simulink model "rlWalkingBipedRobot"  (R2024a)
settings: Solver=ode23t  StartTime=0.0  StopTime=Tf  RelTol=1e-2  EnableMultiTasking=on
values from neighbouring files (symbols this model uses):
  height_plane = 0.025    [robotParametersRL.m]
  init_angs_L = zeros(1,2)    [robotParametersRL.m]    (also in walkerResetFcn.m)
  init_angs_R = zeros(1,2)    [robotParametersRL.m]    (also in walkerResetFcn.m)
  init_height = foot_z + h +                torso_z/2 + torso_offset_z + height_plane/2    (= 21.0125)    [robotParametersRL.m]
  joint_stiffness = 0    [robotParametersRL.m]
  lower_leg_length = 10    [robotParametersRL.m]
  max_torque = 3    [robotParametersRL.m]
  plane_x = 25    [robotParametersRL.m]
  plane_y = 10    [robotParametersRL.m]
  s = load(files(i).name,'trainingStats')    [comparePerformance.m]
  Tf = 10    [robotParametersRL.m]
  torso_offset_x = -1    [robotParametersRL.m]
  torso_offset_z = -2    [robotParametersRL.m]
  torso_x = 5    [robotParametersRL.m]
  torso_y = 8    [robotParametersRL.m]
  torso_z = 8    [robotParametersRL.m]
  Ts = 0.025    [robotParametersRL.m]
  upper_leg_length = 10    [robotParametersRL.m]
  wx0 = 0    [robotParametersRL.m]
  wy0 = 0    [robotParametersRL.m]
undefined symbols (not defined in the file or in its folder): X, Y, Z
libraries: sm_lib x27, nesl_utility x14, walkingRobotUtils x10, simulink x5, rllib x1
settings Model: Creator=The MathWorks, Inc.  LastModifiedBy=Administrator
settings SolverCC: ZeroCrossAlgorithm=Adaptive  AlgebraicLoopSolver=TrustRegion
settings DataIOCC: SaveOutput=off  SignalLogging=off  DSMLogging=off  SaveTime=off  ReturnWorkspaceOutputs=off  OutputTimes=0:0.01:10
settings OptimizationCC: LifeSpan=inf
settings DebuggingCC: MaxConsecutiveZCsMsg=warning  IgnoredZcDiagnostic=none  UnconnectedInputMsg=warning  UnconnectedOutputMsg=warning  UnconnectedLineMsg=warning  AllowSymbolicDim=off  SFUnexpectedBacktrackingDiag=warning  SFNoUnconditionalDefaultTransitionDiag=warning  SFExecutionAtInitializationDiag=none  UnitsInconsistencyMsg=none  ArithmeticOperatorsInVariantConditions=warning
settings ModelReferenceCC: EnableRefExpFcnMdlSchedulingChecks=on
settings SFSimCC: SimUseLocalCustomCode=off  CustomCodeUndefinedFunction=UseInterfaceOnly
settings RTWCC: RTWUseLocalCustomCode=off  GPUComputeCapability=3.5
settings CodeAppCC: StateflowObjectComments=on
settings GRTTargetCC: TargetLangStandard=C89/C90 (ANSI)
settings ConfigComp: CovMetricSettings=dw  CovSaveCumulativeToWorkspaceVar=on  CovSaveSingleToWorkspaceVar=on  CovExternalEMLEnable=off  CovSFcnEnable=off
settings SimscapeCC: SimscapeNormalizeSystem=off  SimscapeLogOpenViewer=on  SimscapeLogLimitData=off  SimscapeLogDataHistory=10000
settings ConfigurationSet: Description=SimMechanics 2G
settings DiagnosticsConfigSet: SimMechanicsRigidlyBoundBlock=none
settings ExplorerConfigSet: InternalSimMechanicsExplorerSettings="<ExplorerConfiguration><canonicalview>default</canonicalview><AnimationSetting><BasePlaybackSpeed>1.0</BasePlaybackSpeed><PlaybackSpeedFactor>1.0</PlaybackSpeedFactor></AnimationSetting><TilePanel><TileInfo><Tiles Columns=\"1\" Count=\"1\" Rows=\"1\"><Column Weight=\"1\"/><Row Weight=\"1\"/><Tile Height=\"1\" Width=\"1\" X=\"0\" Y=\"0\"/></Tiles></TileInfo><SceneInfo><SceneViewer><BGColor><R>0.60000002384185791</R><G>0.60000002384185791</G><B>0.60000002384185791</B></BGColor><Camera><DoPerspective>off</DoPerspective><Position><X>7.18002534815406079</X><Y>-8.21011991112170847</Y><Z>8.33180938462712462</Z></Position><Center><X>1.10741005252516134</X><Y>-0.176829942633513204</Y><Z>0.646464709811595872</Z></Center><Up><X>-0.335329266167064488</X><Y>0.506481739462631531</Y><Z>0.79437430147428989</Z></Up><ViewLimDist>1</ViewLimDist><YLim>0.739205014828661411</YLim><XLim>1.12849377732657596</XLim></Camera></SceneViewer></SceneInfo></TilePanel><MechEditorPanel><Cameras/><GfxPanelCameraMap/><VideoCreator><PlaybackSpeedRatio>1.0</PlaybackSpeedRatio><FrameRate>30</FrameRate><VideoFormat>Motion JPEG AVI</VideoFormat><FrameSize>auto</FrameSize></VideoCreator></MechEditorPanel></ExplorerConfiguration>"

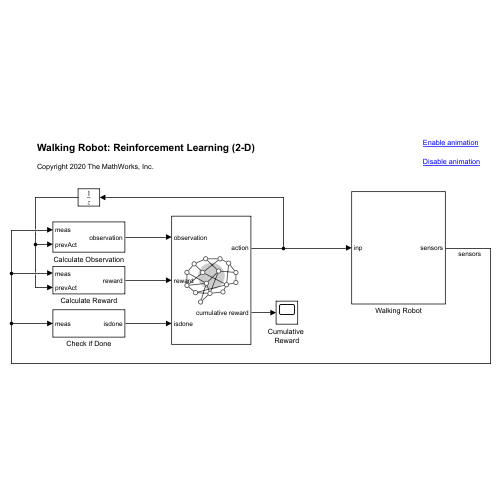
[thumbnail: Simulink's stored preview of the top-level diagram]
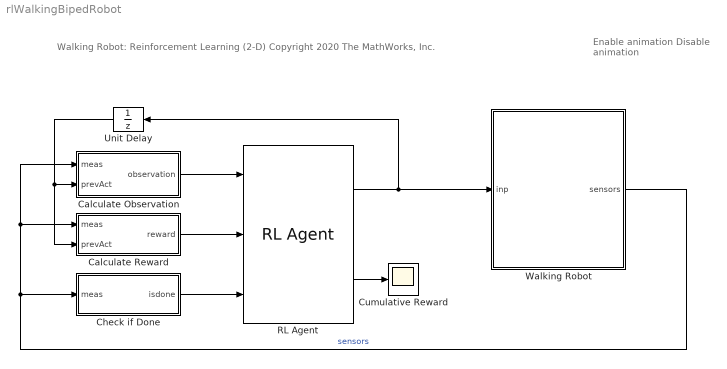
== system rlWalkingBipedRobot ==
  note: Enable animation
      |
      | Disable animation
  note: Walking Robot: Reinforcement Learning (2-D)
      |
      | Copyright 2020 The MathWorks, Inc.
  Calculate Observation : Subsystem
  Calculate Reward : Subsystem
  Check if Done : Subsystem
  Cumulative Reward : Scope
  RL Agent : rllib/RL Agent  Agent=agent  ExternalActionAsInput=off  ProvideLastAction=off  ProvideCumRwd=on  TreatAsDirectFeedthrough=on  UseStrictObservationDataTypes=off
  Unit Delay : UnitDelay  SampleTime=-1  HasFrameUpgradeWarning=on
  Walking Robot : Subsystem
  wires:
  Walking Robot/1(sensors) -> Calculate Reward/1(meas), Calculate Observation/1(meas), Check if Done/1(meas)  "sensors"
  Calculate Reward/1(reward) -> RL Agent/2
  Calculate Observation/1(observation) -> RL Agent/1
  Check if Done/1(isdone) -> RL Agent/3
  RL Agent/2 -> Cumulative Reward/1
  Unit Delay/1 -> Calculate Reward/2(prevAct), Calculate Observation/2(prevAct)
  RL Agent/1 -> Walking Robot/1(inp), Unit Delay/1

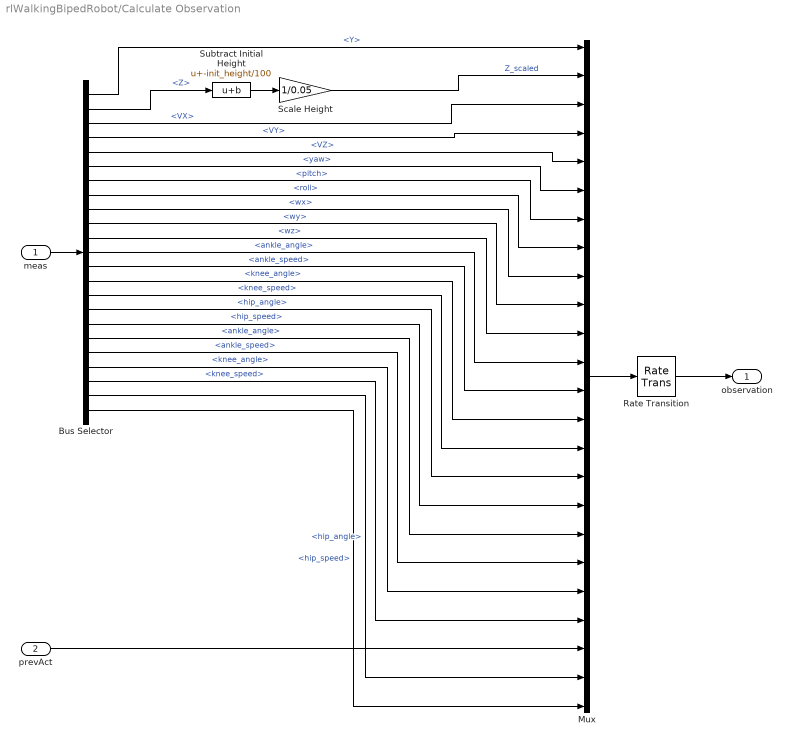
== system rlWalkingBipedRobot/Calculate Observation ==
  meas : Inport
  prevAct : Inport  Port=2
  Bus Selector : BusSelector  OutputSignals=Y,Z,VX,VY,VZ,yaw,pitch,roll,wx,wy,wz,measR.ankle_angle,measR.ankle_speed,measR.knee_angle,measR.knee_speed,measR.hip_angle,measR.hip_speed,measL.ankle_angle,measL.ankle_speed,measL.knee_angle,measL.knee_speed,measL.hip_angle,measL.hip_speed
  Mux : Mux  Inputs=24
  Rate Transition : RateTransition
  Scale Height : Gain  Gain=1/0.05
  Subtract Initial Height : Bias  Bias=-init_height/100  SaturateOnIntegerOverflow=off
  observation : Outport  VectorParamsAs1DForOutWhenUnconnected=off
  wires:
  meas/1 -> Bus Selector/1
  Mux/1 -> Rate Transition/1
  Rate Transition/1 -> observation/1
  prevAct/1 -> Mux/22
  Bus Selector/2 -> Subtract Initial Height/1  "<Z>"
  Subtract Initial Height/1 -> Scale Height/1
  Scale Height/1 -> Mux/2  "Z_scaled"
  Bus Selector/1 -> Mux/1  "<Y>"
  Bus Selector/4 -> Mux/4  "<VY>"
  Bus Selector/5 -> Mux/5  "<VZ>"
  Bus Selector/3 -> Mux/3  "<VX>"
  Bus Selector/6 -> Mux/6  "<yaw>"
  Bus Selector/7 -> Mux/7  "<pitch>"
  Bus Selector/8 -> Mux/8  "<roll>"
  Bus Selector/9 -> Mux/9  "<wx>"
  Bus Selector/10 -> Mux/10  "<wy>"
  Bus Selector/11 -> Mux/11  "<wz>"
  Bus Selector/12 -> Mux/12  "<ankle_angle>"
  Bus Selector/13 -> Mux/13  "<ankle_speed>"
  Bus Selector/14 -> Mux/14  "<knee_angle>"
  Bus Selector/15 -> Mux/15  "<knee_speed>"
  Bus Selector/16 -> Mux/16  "<hip_angle>"
  Bus Selector/17 -> Mux/17  "<hip_speed>"
  Bus Selector/18 -> Mux/18  "<ankle_angle>"
  Bus Selector/19 -> Mux/19  "<ankle_speed>"
  Bus Selector/20 -> Mux/20  "<knee_angle>"
  Bus Selector/21 -> Mux/21  "<knee_speed>"
  Bus Selector/22 -> Mux/23  "<hip_angle>"
  Bus Selector/23 -> Mux/24  "<hip_speed>"

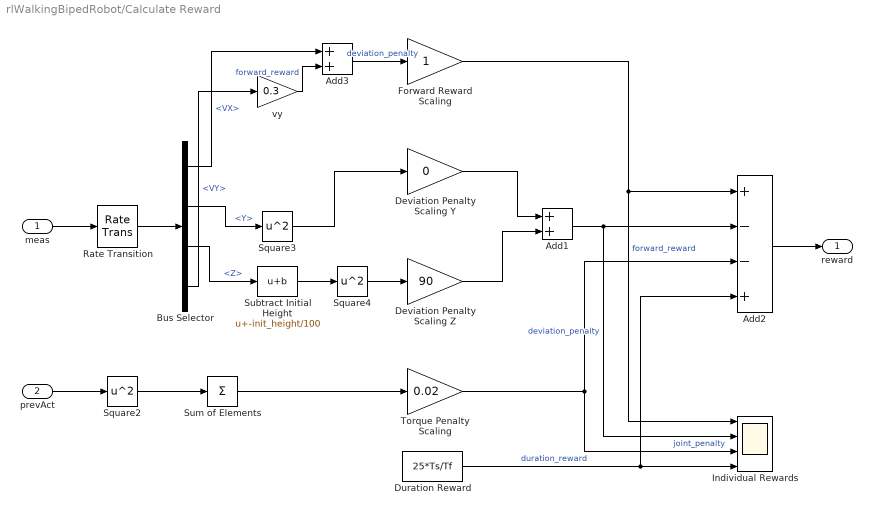
== system rlWalkingBipedRobot/Calculate Reward ==
  meas : Inport
  prevAct : Inport  Port=2
  Add1 : Sum
  Add2 : Sum  Inputs=+--+
  Add3 : Sum
  Bus Selector : BusSelector  OutputSignals=VX,Y,Z,VY
  Deviation Penalty Scaling Y : Gain  Gain=0
  Deviation Penalty Scaling Z : Gain  Gain=90
  Duration Reward : Constant  Value=25*Ts/Tf
  Forward Reward Scaling : Gain
  Individual Rewards : Scope  NumInputPorts=4
  Rate Transition : RateTransition  OutPortSampleTime=Ts
  Square2 : Math  Operator=square  SignedPower=on
  Square3 : Math  Operator=square  SignedPower=on
  Square4 : Math  Operator=square  SignedPower=on
  Subtract Initial Height : Bias  Bias=-init_height/100  SaturateOnIntegerOverflow=off
  Sum of Elements : Sum  Inputs=+
  Torque Penalty Scaling : Gain  Gain=0.02
  vy : Gain  Gain=0.3
  reward : Outport  VectorParamsAs1DForOutWhenUnconnected=off
  wires:
  meas/1 -> Rate Transition/1
  Rate Transition/1 -> Bus Selector/1
  Add2/1 -> reward/1
  Add1/1 -> Add2/2, Individual Rewards/2  "deviation_penalty"
  Forward Reward Scaling/1 -> Add2/1, Individual Rewards/1  "forward_reward"
  Sum of Elements/1 -> Torque Penalty Scaling/1
  Bus Selector/1 -> Add3/1  "<VX>"
  Bus Selector/2 -> Square3/1  "<Y>"
  Square3/1 -> Deviation Penalty Scaling Y/1
  Duration Reward/1 -> Individual Rewards/4, Add2/4  "duration_reward"
  prevAct/1 -> Square2/1
  Square2/1 -> Sum of Elements/1
  Torque Penalty Scaling/1 -> Add2/3, Individual Rewards/3  "joint_penalty"
  Square4/1 -> Deviation Penalty Scaling Z/1
  Bus Selector/3 -> Subtract Initial Height/1  "<Z>"
  Subtract Initial Height/1 -> Square4/1
  Deviation Penalty Scaling Z/1 -> Add1/2
  Deviation Penalty Scaling Y/1 -> Add1/1
  Add3/1 -> Forward Reward Scaling/1  "deviation_penalty"
  vy/1 -> Add3/2  "forward_reward"
  Bus Selector/4 -> vy/1  "<VY>"

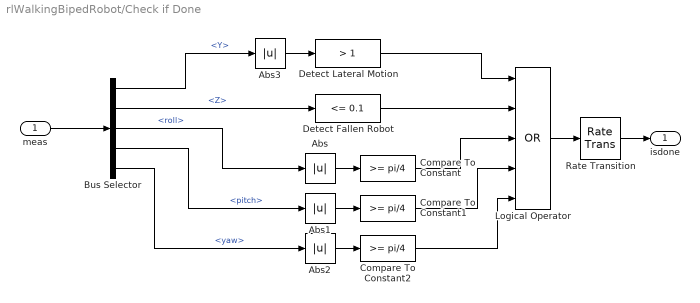
== system rlWalkingBipedRobot/Check if Done ==
  meas : Inport
  Abs{,1..3} (4 alike) : Abs  SaturateOnIntegerOverflow=off
  Bus Selector : BusSelector  OutputSignals=Y,Z,roll,pitch,yaw
  Compare To Constant : simulink/Logic and Bit Operations/Compare To Constant  relop=>=  const=pi/4  OutDataTypeStr=boolean
  Compare To Constant1 : simulink/Logic and Bit Operations/Compare To Constant  relop=>=  const=pi/4  OutDataTypeStr=boolean
  Compare To Constant2 : simulink/Logic and Bit Operations/Compare To Constant  relop=>=  const=pi/4  OutDataTypeStr=boolean
  Detect Fallen Robot : simulink/Logic and Bit Operations/Compare To Constant  relop=<=  const=0.1  OutDataTypeStr=boolean
  Detect Lateral Motion : simulink/Logic and Bit Operations/Compare To Constant  relop=>  const=1  OutDataTypeStr=boolean
  Logical Operator : Logic  Operator=OR  Inputs=5  AllPortsSameDT=off  OutDataTypeStr=boolean
  Rate Transition : RateTransition
  isdone : Outport  VectorParamsAs1DForOutWhenUnconnected=off
  wires:
  Logical Operator/1 -> Rate Transition/1
  Bus Selector/2 -> Detect Fallen Robot/1  "<Z>"
  meas/1 -> Bus Selector/1
  Detect Fallen Robot/1 -> Logical Operator/2
  Bus Selector/3 -> Abs/1  "<roll>"
  Bus Selector/4 -> Abs1/1  "<pitch>"
  Compare To Constant/1 -> Logical Operator/3
  Abs/1 -> Compare To Constant/1
  Abs1/1 -> Compare To Constant1/1
  Compare To Constant1/1 -> Logical Operator/4
  Rate Transition/1 -> isdone/1
  Abs2/1 -> Compare To Constant2/1
  Bus Selector/5 -> Abs2/1  "<yaw>"
  Compare To Constant2/1 -> Logical Operator/5
  Abs3/1 -> Detect Lateral Motion/1
  Bus Selector/1 -> Abs3/1  "<Y>"
  Detect Lateral Motion/1 -> Logical Operator/1

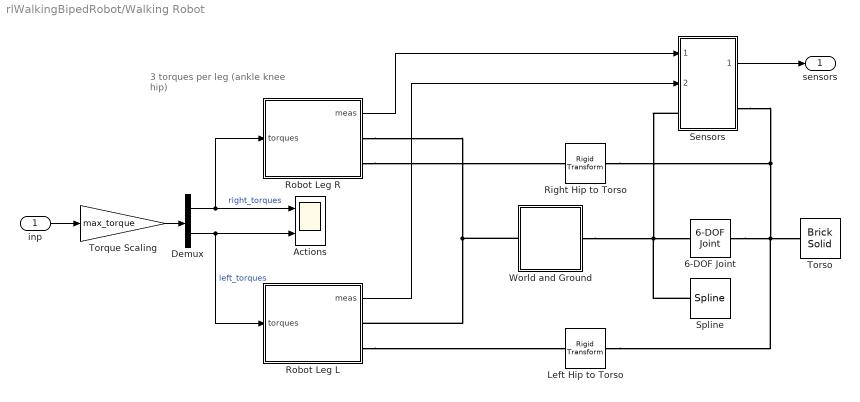
== system rlWalkingBipedRobot/Walking Robot ==
  note: 3 torques per leg
      | (ankle knee hip)
  inp : Inport
  6-DOF Joint : sm_lib/Joints/6-DOF Joint  JointMode=Normal  CompositeWrenchDir=FollowerOnBase  CompositeWrenchFrame=BaseFrame  SenseConstraintForce=off  SenseConstraintTorque=off  SenseTotalForce=off  SenseTotalTorque=off  PxPositionTargetSpecify=on  PxPositionTargetPriority=High  PxPositionTargetValue=0  PxPositionTargetValueUnits=m  PxVelocityTargetSpecify=on  PxVelocityTargetPriority=High  PxVelocityTargetValue=vx0  PxVelocityTargetValueUnits=m/s  PxEquilibriumPosition=0  PxEquilibriumPositionUnits=m  PxSpringStiffness=0  PxSpringStiffnessUnits=N/m  PxDampingCoefficient=world_damping  PxDampingCoefficientUnits=N/(m/s)  PxLowerLimitSpecify=off  PxLowerLimitBound=-1  PxLowerLimitBoundUnits=m  PxLowerLimitStiffness=1e6  PxLowerLimitStiffnessUnits=N/m  PxLowerLimitDamping=1e3  PxLowerLimitDampingUnits=N/(m/s)  PxLowerLimitTransitionRegionWidth=1e-4  PxLowerLimitTransitionRegionWidthUnits=m  PxUpperLimitSpecify=off  PxUpperLimitBound=1  PxUpperLimitBoundUnits=m  PxUpperLimitStiffness=1e6  PxUpperLimitStiffnessUnits=N/m  PxUpperLimitDamping=1e3  PxUpperLimitDampingUnits=N/(m/s)  PxUpperLimitTransitionRegionWidth=1e-4  PxUpperLimitTransitionRegionWidthUnits=m  PxTorqueActuationMode=NoTorque  PxMotionActuationMode=ComputedMotion  PxSensePosition=off  PxSenseVelocity=off  PxSenseAcceleration=off  PxSenseTorqueForce=off  PxSenseLowerLimitTorqueForce=off  PxSenseUpperLimitTorqueForce=off  PyPositionTargetSpecify=on  PyPositionTargetPriority=High  PyPositionTargetValue=0  PyPositionTargetValueUnits=m  PyVelocityTargetSpecify=on  PyVelocityTargetPriority=High  PyVelocityTargetValue=0  PyVelocityTargetValueUnits=m/s  PyEquilibriumPosition=0  PyEquilibriumPositionUnits=m  PySpringStiffness=0  PySpringStiffnessUnits=N/m  PyDampingCoefficient=world_damping  PyDampingCoefficientUnits=N/(m/s)  PyLowerLimitSpecify=off  PyLowerLimitBound=-1  PyLowerLimitBoundUnits=m  PyLowerLimitStiffness=1e6  PyLowerLimitStiffnessUnits=N/m  PyLowerLimitDamping=1e3  PyLowerLimitDampingUnits=N/(m/s)  PyLowerLimitTransitionRegionWidth=1e-4  PyLowerLimitTransitionRegionWidthUnits=m  PyUpperLimitSpecify=off  PyUpperLimitBound=1  PyUpperLimitBoundUnits=m  PyUpperLimitStiffness=1e6  PyUpperLimitStiffnessUnits=N/m  PyUpperLimitDamping=1e3  PyUpperLimitDampingUnits=N/(m/s)  PyUpperLimitTransitionRegionWidth=1e-4  PyUpperLimitTransitionRegionWidthUnits=m  PyTorqueActuationMode=NoTorque  PyMotionActuationMode=ComputedMotion  PySensePosition=off  PySenseVelocity=off  PySenseAcceleration=off  PySenseTorqueForce=off  PySenseLowerLimitTorqueForce=off  PySenseUpperLimitTorqueForce=off  PzPositionTargetSpecify=on  PzPositionTargetPriority=High  PzPositionTargetValue=init_height  PzPositionTargetValueUnits=cm  PzVelocityTargetSpecify=off  PzVelocityTargetPriority=High  PzVelocityTargetValue=0  PzVelocityTargetValueUnits=m/s  PzEquilibriumPosition=0  PzEquilibriumPositionUnits=m  PzSpringStiffness=0  PzSpringStiffnessUnits=N/m  PzDampingCoefficient=world_damping  PzDampingCoefficientUnits=N/(m/s)  PzLowerLimitSpecify=off  PzLowerLimitBound=-1  PzLowerLimitBoundUnits=m  PzLowerLimitStiffness=1e6  PzLowerLimitStiffnessUnits=N/m  PzLowerLimitDamping=1e3  PzLowerLimitDampingUnits=N/(m/s)  PzLowerLimitTransitionRegionWidth=1e-4  PzLowerLimitTransitionRegionWidthUnits=m  PzUpperLimitSpecify=off  PzUpperLimitBound=1  PzUpperLimitBoundUnits=m  PzUpperLimitStiffness=1e6  PzUpperLimitStiffnessUnits=N/m  PzUpperLimitDamping=1e3  PzUpperLimitDampingUnits=N/(m/s)  PzUpperLimitTransitionRegionWidth=1e-4  PzUpperLimitTransitionRegionWidthUnits=m  PzTorqueActuationMode=NoTorque  PzMotionActuationMode=ComputedMotion  PzSensePosition=off  PzSenseVelocity=off  PzSenseAcceleration=off  PzSenseTorqueForce=off  PzSenseLowerLimitTorqueForce=off  PzSenseUpperLimitTorqueForce=off  SphPositionTargetSpecify=on  SphPositionTargetPriority=High  SphPositionTargetRotationMethod=RotationSequence  SphPositionTargetFollAlignAxisA=+X  SphPositionTargetBaseAlignAxisA=+Y  SphPositionTargetFollAlignAxisB=+Y  SphPositionTargetBaseAlignAxisB=+Z  SphPositionTargetRotationStandardAxis=+Z  SphPositionTargetRotationAngle=0.0  SphPositionTargetRotationAngleUnits=deg  SphPositionTargetRotationArbitraryAxis=[0 0 1]  SphPositionTargetRotationSequenceAxes=FollowerAxes  SphPositionTargetRotationSequence=XYX  SphPositionTargetRotationSequenceAngles=[wx0 wy0 0]  SphPositionTargetRotationSequenceAnglesUnits=rad  SphPositionTargetRotationMatrix=eye(3)  SphPositionTargetQuaternion=[1 0 0 0]  SphVelocityTargetSpecify=off  SphVelocityTargetPriority=High  SphVelocityTargetValue=[0 0 0]  SphVelocityTargetValueUnits=deg/s  SphVelocityTargetInFollowerFrame=on  SphEqPosRotationMethod=None  SphEqPosFollAlignAxisA=+X  SphEqPosBaseAlignAxisA=+Y  SphEqPosFollAlignAxisB=+Y  SphEqPosBaseAlignAxisB=+Z  SphEqPosRotationStandardAxis=+Z  SphEqPosRotationAngle=0.0  SphEqPosRotationAngleUnits=deg  SphEqPosRotationArbitraryAxis=[0 0 1]  SphEqPosRotationSequenceAxes=FollowerAxes  SphEqPosRotationSequence=XYX  SphEqPosRotationSequenceAngles=[0 0 0]  SphEqPosRotationSequenceAnglesUnits=deg  SphEqPosRotationMatrix=[1 0 0; 0 1 0; 0 0 1]  SphEqPosQuaternion=[1 0 0 0]  SphSpringStiffness=0  SphSpringStiffnessUnits=N*m/deg  SphDampingCoefficient=world_rot_damping  SphDampingCoefficientUnits=N*m/(rad/s)  SphLowerLimitSpecify=off  SphLowerLimitBound=15  SphLowerLimitBoundUnits=deg  SphLowerLimitStiffness=1e4  SphLowerLimitStiffnessUnits=N*m/deg  SphLowerLimitDamping=10  SphLowerLimitDampingUnits=N*m/(deg/s)  SphLowerLimitTransitionRegionWidth=0.1  SphLowerLimitTransitionRegionWidthUnits=deg  SphUpperLimitSpecify=off  SphUpperLimitBound=45  SphUpperLimitBoundUnits=deg  SphUpperLimitStiffness=1e4  SphUpperLimitStiffnessUnits=N*m/deg  SphUpperLimitDamping=10  SphUpperLimitDampingUnits=N*m/(deg/s)  SphUpperLimitTransitionRegionWidth=0.1  SphUpperLimitTransitionRegionWidthUnits=deg  SphTorqueActuationMode=NoTorque  SphActuateTorqueX=off  SphActuateTorqueY=off  SphActuateTorqueZ=off  SphActuateTorque=off  SphActuationFrame=BaseFrame  SphSensePosition=off  SphSenseVelocityX=off  SphSenseVelocityY=off  SphSenseVelocityZ=off  SphSenseVelocity=off  SphSenseAccelerationX=off  SphSenseAccelerationY=off  SphSenseAccelerationZ=off  SphSenseAcceleration=off  SphSenseLowerLimitTorqueMag=off  SphSenseUpperLimitTorqueMag=off  SphSensingFrame=BaseFrame
  Actions : Scope  NumInputPorts=2
  Demux : Demux  Outputs=2
  Left Hip to Torso : sm_lib/Frames and Transforms/Rigid Transform  RotationMethod=None  FollAlignAxisA=+X  BaseAlignAxisA=+Y  FollAlignAxisB=+Y  BaseAlignAxisB=+Z  RotationStandardAxis=+Z  RotationAngle=0.0  RotationAngleUnits=deg  RotationArbitraryAxis=[0 0 1]  RotationSequenceAxes=FollowerAxes  RotationSequence=XYX  RotationSequenceAngles=[0 0 0]  RotationSequenceAnglesUnits=deg  RotationMatrix=[1 0 0; 0 1 0; 0 0 1]  Quaternion=[1 0 0 0]  TranslationMethod=Cartesian  TranslationCartesianOffset=[torso_offset_x torso_y/2 torso_offset_z]  TranslationCartesianOffsetUnits=cm  TranslationStandardAxis=+Z  TranslationStandardOffset=0  TranslationStandardOffsetUnits=cm  TranslationROffset=0  TranslationROffsetUnits=m  TranslationThetaOffset=0  TranslationThetaOffsetUnits=deg  TranslationZOffset=0  TranslationZOffsetUnits=m
  Right Hip to Torso : sm_lib/Frames and Transforms/Rigid Transform  RotationMethod=None  FollAlignAxisA=+X  BaseAlignAxisA=+Y  FollAlignAxisB=+Y  BaseAlignAxisB=+Z  RotationStandardAxis=+Z  RotationAngle=0.0  RotationAngleUnits=deg  RotationArbitraryAxis=[0 0 1]  RotationSequenceAxes=FollowerAxes  RotationSequence=XYX  RotationSequenceAngles=[0 0 0]  RotationSequenceAnglesUnits=deg  RotationMatrix=[1 0 0; 0 1 0; 0 0 1]  Quaternion=[1 0 0 0]  TranslationMethod=Cartesian  TranslationCartesianOffset=[torso_offset_x -torso_y/2 torso_offset_z]  TranslationCartesianOffsetUnits=cm  TranslationStandardAxis=+Z  TranslationStandardOffset=0  TranslationStandardOffsetUnits=cm  TranslationROffset=0  TranslationROffsetUnits=m  TranslationThetaOffset=0  TranslationThetaOffsetUnits=deg  TranslationZOffset=0  TranslationZOffsetUnits=m
  Robot Leg L : Subsystem
  Robot Leg R : Subsystem
  Sensors : Subsystem
  Spline : sm_lib/Curves and Surfaces/Spline  DataPoints=[0 0 0.025; 5 0 0.025]  DataPointsUnits=m  EndConditionType=Natural  GraphicType=FromGeometry  MarkerShape=Sphere  MarkerSize=10  GraphicVisPropType=SimpleVisualProperties  GraphicDiffuseColor=[0 0 0]  GraphicOpacity=1.0  GraphicSpecularColor=[0.5 0.5 0.5 1.0]  GraphicAmbientColor=[0.15 0.15 0.15 1.0]  GraphicEmissiveColor=[0.0 0.0 0.0 1.0]  GraphicShininess=75
  Torque Scaling : Gain  Gain=max_torque
  Torso : sm_lib/Body Elements/Brick Solid  BrickDimensions=[torso_x torso_y torso_z]  BrickDimensionsUnits=cm  ExportEntireGeometry=off  InertiaType=CalculateFromGeometry  BasedOnType=Density  Density=density  DensityUnits=kg/m^3  Mass=1  MassUnits=kg  CenterOfMass=[0 0 0]  CenterOfMassUnits=m  MomentsOfInertia=[1 1 1]  MomentsOfInertiaUnits=kg*m^2  ProductsOfInertia=[1 1 1]  ProductsOfInertiaUnits=kg*m^2  GraphicType=FromGeometry  MarkerShape=Sphere  MarkerSize=10  GraphicVisPropType=SimpleVisualProperties  GraphicDiffuseColor=[0.5 0.5 0.5]  GraphicOpacity=1.0  GraphicSpecularColor=[0.5 0.5 0.5 1.0]  GraphicAmbientColor=[0.15 0.15 0.15 1.0]  GraphicEmissiveColor=[0.0 0.0 0.0 1.0]  GraphicShininess=75  DoExposeReferenceFrame=on  SerializedFrames=<Frames/>
  World and Ground : Subsystem
  sensors : Outport  VectorParamsAs1DForOutWhenUnconnected=off
  wires:
  Robot Leg L/1(meas) -> Sensors/2(measL)
  Robot Leg R/1(meas) -> Sensors/1(measR)
  Sensors/1(sensors) -> sensors/1
  inp/1 -> Torque Scaling/1
  Demux/2 -> Robot Leg L/1(torques), Actions/2  "left_torques"
  Demux/1 -> Robot Leg R/1(torques), Actions/1  "right_torques"
  Torque Scaling/1 -> Demux/1
  connections:
  Robot Leg R/RConn2 -- Right Hip to Torso/RConn1
  Robot Leg L/RConn2 -- Left Hip to Torso/RConn1
  Right Hip to Torso/LConn1 -- Sensors/RConn1 -- Left Hip to Torso/LConn1 -- Torso/RConn1 -- 6-DOF Joint/RConn1
  Spline/LConn1 -- World and Ground/LConn1 -- Sensors/LConn1 -- 6-DOF Joint/LConn1
  World and Ground/RConn1 -- Robot Leg R/RConn1 -- Robot Leg L/RConn1

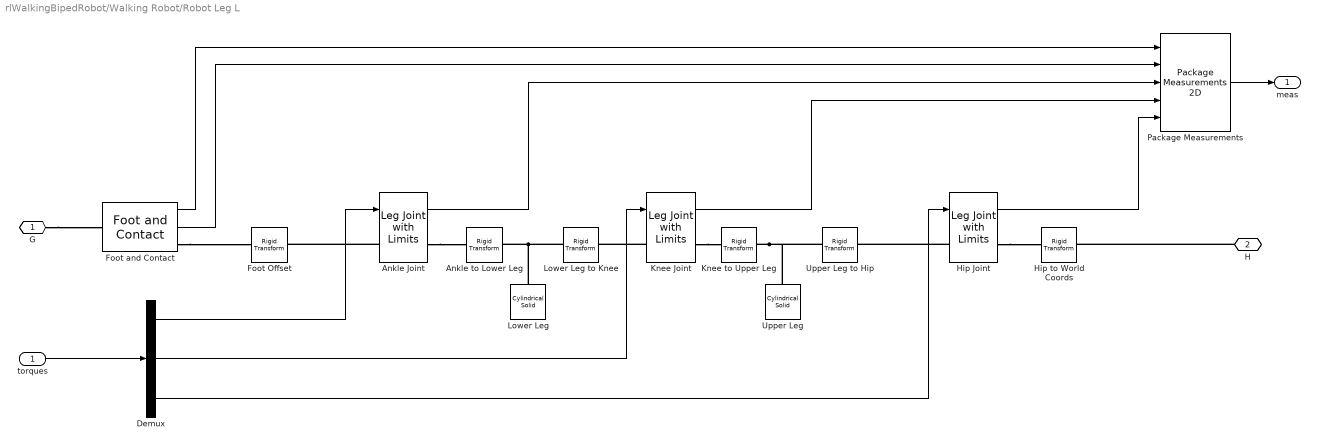
== system rlWalkingBipedRobot/Walking Robot/Robot Leg L ==
  torques : Inport
  Ankle Joint : walkingRobotUtils/Leg Joint with Limits  VariantControl=actuatorType == 2  k=joint_stiffness  d=joint_damping  initAngle=-sum(init_angs_L)  eqAngle=0  upperLimit=pi/4  lowerLimit=-pi/4  jointLimitStiffness=joint_limit_stiffness  jointLimitDamping=joint_limit_damping
  Ankle to Lower Leg : sm_lib/Frames and Transforms/Rigid Transform  RotationMethod=StandardAxis  FollAlignAxisA=+X  BaseAlignAxisA=+Y  FollAlignAxisB=+Y  BaseAlignAxisB=+Z  RotationStandardAxis=+X  RotationAngle=-90  RotationAngleUnits=deg  RotationArbitraryAxis=[0 0 1]  RotationSequenceAxes=FollowerAxes  RotationSequence=XYX  RotationSequenceAngles=[0 0 0]  RotationSequenceAnglesUnits=deg  RotationMatrix=[1 0 0; 0 1 0; 0 0 1]  Quaternion=[1 0 0 0]  TranslationMethod=Cartesian  TranslationCartesianOffset=[0 lower_leg_length/2 0]  TranslationCartesianOffsetUnits=cm  TranslationStandardAxis=+Z  TranslationStandardOffset=0  TranslationStandardOffsetUnits=cm  TranslationROffset=0  TranslationROffsetUnits=m  TranslationThetaOffset=0  TranslationThetaOffsetUnits=deg  TranslationZOffset=0  TranslationZOffsetUnits=m
  Demux : Demux  Outputs=3
  Foot Offset : sm_lib/Frames and Transforms/Rigid Transform  RotationMethod=None  FollAlignAxisA=+X  BaseAlignAxisA=+Y  FollAlignAxisB=+Y  BaseAlignAxisB=+Z  RotationStandardAxis=+X  RotationAngle=-90  RotationAngleUnits=deg  RotationArbitraryAxis=[0 0 1]  RotationSequenceAxes=FollowerAxes  RotationSequence=XYX  RotationSequenceAngles=[0 0 0]  RotationSequenceAnglesUnits=deg  RotationMatrix=[1 0 0; 0 1 0; 0 0 1]  Quaternion=[1 0 0 0]  TranslationMethod=Cartesian  TranslationCartesianOffset=foot_offset  TranslationCartesianOffsetUnits=cm  TranslationStandardAxis=+Z  TranslationStandardOffset=0  TranslationStandardOffsetUnits=cm  TranslationROffset=0  TranslationROffsetUnits=m  TranslationThetaOffset=0  TranslationThetaOffsetUnits=deg  TranslationZOffset=0  TranslationZOffsetUnits=m
  Foot and Contact : walkingRobotUtils/Foot and Contact  SystemSampleTime=-1  VariantActivationTime=update diagram  AllowFlexibleInterface=on  Latency=0  AutoFrameSizeCalculation=off
  Hip Joint : walkingRobotUtils/Leg Joint with Limits  VariantControl=actuatorType == 2  k=joint_stiffness  d=joint_damping  initAngle=init_angs_L(1)  eqAngle=0  upperLimit=pi/4  lowerLimit=-pi/4  jointLimitStiffness=joint_limit_stiffness  jointLimitDamping=joint_limit_damping
  Hip to World Coords : sm_lib/Frames and Transforms/Rigid Transform  RotationMethod=StandardAxis  FollAlignAxisA=+X  BaseAlignAxisA=+Y  FollAlignAxisB=+Y  BaseAlignAxisB=+Z  RotationStandardAxis=+X  RotationAngle=-90  RotationAngleUnits=deg  RotationArbitraryAxis=[0 0 1]  RotationSequenceAxes=FollowerAxes  RotationSequence=XYX  RotationSequenceAngles=[0 0 0]  RotationSequenceAnglesUnits=deg  RotationMatrix=[1 0 0; 0 1 0; 0 0 1]  Quaternion=[1 0 0 0]  TranslationMethod=None  TranslationCartesianOffset=[0 0 upper_leg_length/2]  TranslationCartesianOffsetUnits=cm  TranslationStandardAxis=+Z  TranslationStandardOffset=0  TranslationStandardOffsetUnits=cm  TranslationROffset=0  TranslationROffsetUnits=m  TranslationThetaOffset=0  TranslationThetaOffsetUnits=deg  TranslationZOffset=0  TranslationZOffsetUnits=m
  Knee Joint : walkingRobotUtils/Leg Joint with Limits  VariantControl=actuatorType == 2  k=joint_stiffness  d=joint_damping  initAngle=init_angs_L(2)  eqAngle=0  upperLimit=pi  lowerLimit=0  jointLimitStiffness=joint_limit_stiffness  jointLimitDamping=joint_limit_damping
  Knee to Upper Leg : sm_lib/Frames and Transforms/Rigid Transform  RotationMethod=StandardAxis  FollAlignAxisA=+X  BaseAlignAxisA=+Y  FollAlignAxisB=+Y  BaseAlignAxisB=+Z  RotationStandardAxis=+X  RotationAngle=-90  RotationAngleUnits=deg  RotationArbitraryAxis=[0 0 1]  RotationSequenceAxes=FollowerAxes  RotationSequence=XYX  RotationSequenceAngles=[0 0 0]  RotationSequenceAnglesUnits=deg  RotationMatrix=[1 0 0; 0 1 0; 0 0 1]  Quaternion=[1 0 0 0]  TranslationMethod=Cartesian  TranslationCartesianOffset=[0 upper_leg_length/2 0]  TranslationCartesianOffsetUnits=cm  TranslationStandardAxis=+Z  TranslationStandardOffset=0  TranslationStandardOffsetUnits=cm  TranslationROffset=0  TranslationROffsetUnits=m  TranslationThetaOffset=0  TranslationThetaOffsetUnits=deg  TranslationZOffset=0  TranslationZOffsetUnits=m
  Lower Leg : sm_lib/Body Elements/Cylindrical Solid  CylinderRadius=leg_radius  CylinderRadiusUnits=cm  CylinderLength=lower_leg_length  CylinderLengthUnits=cm  ExportEntireGeometry=off  InertiaType=CalculateFromGeometry  BasedOnType=Density  Density=density  DensityUnits=kg/m^3  Mass=1  MassUnits=kg  CenterOfMass=[0 0 0]  CenterOfMassUnits=m  MomentsOfInertia=[1 1 1]  MomentsOfInertiaUnits=kg*m^2  ProductsOfInertia=[1 1 1]  ProductsOfInertiaUnits=kg*m^2  GraphicType=FromGeometry  MarkerShape=Sphere  MarkerSize=10  GraphicVisPropType=SimpleVisualProperties  GraphicDiffuseColor=[0.4 0.4 1.0]  GraphicOpacity=1.0  GraphicSpecularColor=[0.5 0.5 0.5 1.0]  GraphicAmbientColor=[0.15 0.15 0.15 1.0]  GraphicEmissiveColor=[0.0 0.0 0.0 1.0]  GraphicShininess=75  DoExposeReferenceFrame=on  SerializedFrames=<Frames/>
  Lower Leg to Knee : sm_lib/Frames and Transforms/Rigid Transform  RotationMethod=StandardAxis  FollAlignAxisA=+X  BaseAlignAxisA=+Y  FollAlignAxisB=+Y  BaseAlignAxisB=+Z  RotationStandardAxis=+X  RotationAngle=90  RotationAngleUnits=deg  RotationArbitraryAxis=[0 0 1]  RotationSequenceAxes=FollowerAxes  RotationSequence=XYX  RotationSequenceAngles=[0 0 0]  RotationSequenceAnglesUnits=deg  RotationMatrix=[1 0 0; 0 1 0; 0 0 1]  Quaternion=[1 0 0 0]  TranslationMethod=Cartesian  TranslationCartesianOffset=[0 0 lower_leg_length/2]  TranslationCartesianOffsetUnits=cm  TranslationStandardAxis=+Z  TranslationStandardOffset=0  TranslationStandardOffsetUnits=cm  TranslationROffset=0  TranslationROffsetUnits=m  TranslationThetaOffset=0  TranslationThetaOffsetUnits=deg  TranslationZOffset=0  TranslationZOffsetUnits=m
  Package Measurements : walkingRobotUtils/Package  Measurements 2D  SystemSampleTime=-1  VariantActivationTime=update diagram  AllowFlexibleInterface=on  Latency=0  AutoFrameSizeCalculation=off
  Upper Leg : sm_lib/Body Elements/Cylindrical Solid  CylinderRadius=leg_radius  CylinderRadiusUnits=cm  CylinderLength=upper_leg_length  CylinderLengthUnits=cm  ExportEntireGeometry=off  InertiaType=CalculateFromGeometry  BasedOnType=Density  Density=density  DensityUnits=kg/m^3  Mass=1  MassUnits=kg  CenterOfMass=[0 0 0]  CenterOfMassUnits=m  MomentsOfInertia=[1 1 1]  MomentsOfInertiaUnits=kg*m^2  ProductsOfInertia=[1 1 1]  ProductsOfInertiaUnits=kg*m^2  GraphicType=FromGeometry  MarkerShape=Sphere  MarkerSize=10  GraphicVisPropType=SimpleVisualProperties  GraphicDiffuseColor=[1.0 0.4 0.4]  GraphicOpacity=1.0  GraphicSpecularColor=[0.5 0.5 0.5 1.0]  GraphicAmbientColor=[0.15 0.15 0.15 1.0]  GraphicEmissiveColor=[0.0 0.0 0.0 1.0]  GraphicShininess=75  DoExposeReferenceFrame=on  SerializedFrames=<Frames/>
  Upper Leg to Hip : sm_lib/Frames and Transforms/Rigid Transform  RotationMethod=StandardAxis  FollAlignAxisA=+X  BaseAlignAxisA=+Y  FollAlignAxisB=+Y  BaseAlignAxisB=+Z  RotationStandardAxis=+X  RotationAngle=90  RotationAngleUnits=deg  RotationArbitraryAxis=[0 0 1]  RotationSequenceAxes=FollowerAxes  RotationSequence=XYX  RotationSequenceAngles=[0 0 0]  RotationSequenceAnglesUnits=deg  RotationMatrix=[1 0 0; 0 1 0; 0 0 1]  Quaternion=[1 0 0 0]  TranslationMethod=Cartesian  TranslationCartesianOffset=[0 0 upper_leg_length/2]  TranslationCartesianOffsetUnits=cm  TranslationStandardAxis=+Z  TranslationStandardOffset=0  TranslationStandardOffsetUnits=cm  TranslationROffset=0  TranslationROffsetUnits=m  TranslationThetaOffset=0  TranslationThetaOffsetUnits=deg  TranslationZOffset=0  TranslationZOffsetUnits=m
  G : PMIOPort  Side=Right
  H : PMIOPort  Port=2  Side=Right
  meas : Outport  VectorParamsAs1DForOutWhenUnconnected=off
  wires:
  Foot and Contact/1 -> Package Measurements/1
  Foot and Contact/2 -> Package Measurements/2
  Package Measurements/1 -> meas/1
  torques/1 -> Demux/1
  Hip Joint/1 -> Package Measurements/5
  Knee Joint/1 -> Package Measurements/4
  Ankle Joint/1 -> Package Measurements/3
  Demux/1 -> Ankle Joint/1
  Demux/2 -> Knee Joint/1
  Demux/3 -> Hip Joint/1
  connections:
  Foot and Contact/RConn1 -- Foot Offset/LConn1
  H/RConn1 -- Hip to World Coords/RConn1
  Knee Joint/LConn1 -- Lower Leg to Knee/RConn1
  Knee to Upper Leg/RConn1 -- Upper Leg/RConn1 -- Upper Leg to Hip/LConn1
  Lower Leg to Knee/LConn1 -- Lower Leg/RConn1 -- Ankle to Lower Leg/RConn1
  G/RConn1 -- Foot and Contact/LConn1
  Knee Joint/RConn1 -- Knee to Upper Leg/LConn1
  Ankle Joint/RConn1 -- Ankle to Lower Leg/LConn1
  Hip Joint/RConn1 -- Hip to World Coords/LConn1
  Ankle Joint/LConn1 -- Foot Offset/RConn1
  Hip Joint/LConn1 -- Upper Leg to Hip/RConn1

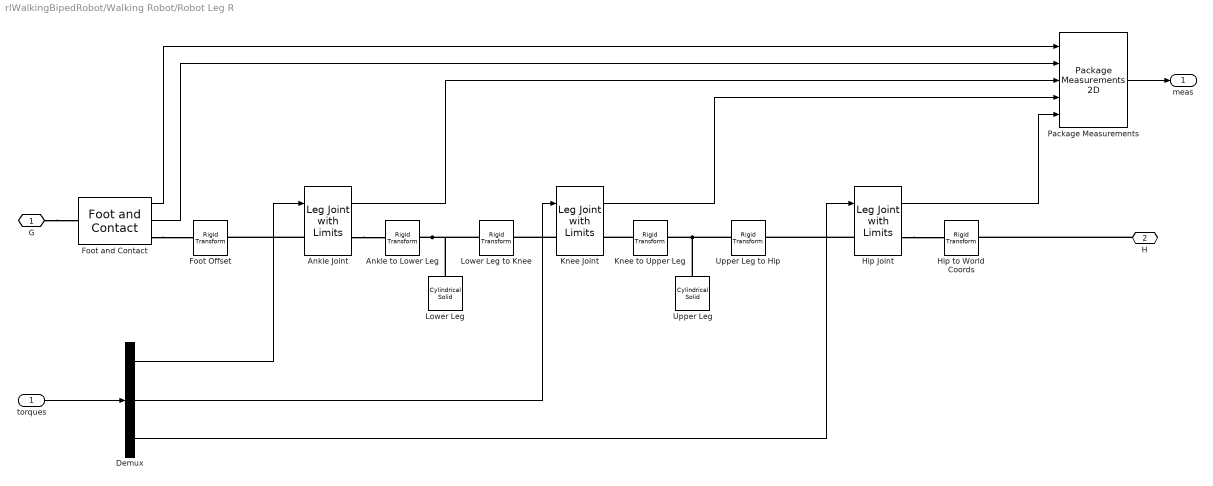
== system rlWalkingBipedRobot/Walking Robot/Robot Leg R ==
  torques : Inport
  Ankle Joint : walkingRobotUtils/Leg Joint with Limits  VariantControl=actuatorType == 2  k=joint_stiffness  d=joint_damping  initAngle=-sum(init_angs_R)  eqAngle=0  upperLimit=pi/4  lowerLimit=-pi/4  jointLimitStiffness=joint_limit_stiffness  jointLimitDamping=joint_limit_damping
  Ankle to Lower Leg : sm_lib/Frames and Transforms/Rigid Transform  RotationMethod=StandardAxis  FollAlignAxisA=+X  BaseAlignAxisA=+Y  FollAlignAxisB=+Y  BaseAlignAxisB=+Z  RotationStandardAxis=+X  RotationAngle=-90  RotationAngleUnits=deg  RotationArbitraryAxis=[0 0 1]  RotationSequenceAxes=FollowerAxes  RotationSequence=XYX  RotationSequenceAngles=[0 0 0]  RotationSequenceAnglesUnits=deg  RotationMatrix=[1 0 0; 0 1 0; 0 0 1]  Quaternion=[1 0 0 0]  TranslationMethod=Cartesian  TranslationCartesianOffset=[0 lower_leg_length/2 0]  TranslationCartesianOffsetUnits=cm  TranslationStandardAxis=+Z  TranslationStandardOffset=0  TranslationStandardOffsetUnits=cm  TranslationROffset=0  TranslationROffsetUnits=m  TranslationThetaOffset=0  TranslationThetaOffsetUnits=deg  TranslationZOffset=0  TranslationZOffsetUnits=m
  Demux : Demux  Outputs=3
  Foot Offset : sm_lib/Frames and Transforms/Rigid Transform  RotationMethod=None  FollAlignAxisA=+X  BaseAlignAxisA=+Y  FollAlignAxisB=+Y  BaseAlignAxisB=+Z  RotationStandardAxis=+X  RotationAngle=-90  RotationAngleUnits=deg  RotationArbitraryAxis=[0 0 1]  RotationSequenceAxes=FollowerAxes  RotationSequence=XYX  RotationSequenceAngles=[0 0 0]  RotationSequenceAnglesUnits=deg  RotationMatrix=[1 0 0; 0 1 0; 0 0 1]  Quaternion=[1 0 0 0]  TranslationMethod=Cartesian  TranslationCartesianOffset=foot_offset  TranslationCartesianOffsetUnits=cm  TranslationStandardAxis=+Z  TranslationStandardOffset=0  TranslationStandardOffsetUnits=cm  TranslationROffset=0  TranslationROffsetUnits=m  TranslationThetaOffset=0  TranslationThetaOffsetUnits=deg  TranslationZOffset=0  TranslationZOffsetUnits=m
  Foot and Contact : walkingRobotUtils/Foot and Contact  SystemSampleTime=-1  VariantActivationTime=update diagram  AllowFlexibleInterface=on  Latency=0  AutoFrameSizeCalculation=off
  Hip Joint : walkingRobotUtils/Leg Joint with Limits  VariantControl=actuatorType == 2  k=joint_stiffness  d=joint_damping  initAngle=init_angs_R(1)  eqAngle=0  upperLimit=pi/4  lowerLimit=-pi/4  jointLimitStiffness=joint_limit_stiffness  jointLimitDamping=joint_limit_damping
  Hip to World Coords : sm_lib/Frames and Transforms/Rigid Transform  RotationMethod=StandardAxis  FollAlignAxisA=+X  BaseAlignAxisA=+Y  FollAlignAxisB=+Y  BaseAlignAxisB=+Z  RotationStandardAxis=+X  RotationAngle=-90  RotationAngleUnits=deg  RotationArbitraryAxis=[0 0 1]  RotationSequenceAxes=FollowerAxes  RotationSequence=XYX  RotationSequenceAngles=[0 0 0]  RotationSequenceAnglesUnits=deg  RotationMatrix=[1 0 0; 0 1 0; 0 0 1]  Quaternion=[1 0 0 0]  TranslationMethod=None  TranslationCartesianOffset=[0 0 upper_leg_length/2]  TranslationCartesianOffsetUnits=cm  TranslationStandardAxis=+Z  TranslationStandardOffset=0  TranslationStandardOffsetUnits=cm  TranslationROffset=0  TranslationROffsetUnits=m  TranslationThetaOffset=0  TranslationThetaOffsetUnits=deg  TranslationZOffset=0  TranslationZOffsetUnits=m
  Knee Joint : walkingRobotUtils/Leg Joint with Limits  VariantControl=actuatorType == 2  k=joint_stiffness  d=joint_damping  initAngle=init_angs_R(2)  eqAngle=0  upperLimit=pi  lowerLimit=0  jointLimitStiffness=joint_limit_stiffness  jointLimitDamping=joint_limit_damping
  Knee to Upper Leg : sm_lib/Frames and Transforms/Rigid Transform  RotationMethod=StandardAxis  FollAlignAxisA=+X  BaseAlignAxisA=+Y  FollAlignAxisB=+Y  BaseAlignAxisB=+Z  RotationStandardAxis=+X  RotationAngle=-90  RotationAngleUnits=deg  RotationArbitraryAxis=[0 0 1]  RotationSequenceAxes=FollowerAxes  RotationSequence=XYX  RotationSequenceAngles=[0 0 0]  RotationSequenceAnglesUnits=deg  RotationMatrix=[1 0 0; 0 1 0; 0 0 1]  Quaternion=[1 0 0 0]  TranslationMethod=Cartesian  TranslationCartesianOffset=[0 upper_leg_length/2 0]  TranslationCartesianOffsetUnits=cm  TranslationStandardAxis=+Z  TranslationStandardOffset=0  TranslationStandardOffsetUnits=cm  TranslationROffset=0  TranslationROffsetUnits=m  TranslationThetaOffset=0  TranslationThetaOffsetUnits=deg  TranslationZOffset=0  TranslationZOffsetUnits=m
  Lower Leg : sm_lib/Body Elements/Cylindrical Solid  CylinderRadius=leg_radius  CylinderRadiusUnits=cm  CylinderLength=lower_leg_length  CylinderLengthUnits=cm  ExportEntireGeometry=off  InertiaType=CalculateFromGeometry  BasedOnType=Density  Density=density  DensityUnits=kg/m^3  Mass=1  MassUnits=kg  CenterOfMass=[0 0 0]  CenterOfMassUnits=m  MomentsOfInertia=[1 1 1]  MomentsOfInertiaUnits=kg*m^2  ProductsOfInertia=[1 1 1]  ProductsOfInertiaUnits=kg*m^2  GraphicType=FromGeometry  MarkerShape=Sphere  MarkerSize=10  GraphicVisPropType=SimpleVisualProperties  GraphicDiffuseColor=[0.4 0.4 1.0]  GraphicOpacity=1.0  GraphicSpecularColor=[0.5 0.5 0.5 1.0]  GraphicAmbientColor=[0.15 0.15 0.15 1.0]  GraphicEmissiveColor=[0.0 0.0 0.0 1.0]  GraphicShininess=75  DoExposeReferenceFrame=on  SerializedFrames=<Frames/>
  Lower Leg to Knee : sm_lib/Frames and Transforms/Rigid Transform  RotationMethod=StandardAxis  FollAlignAxisA=+X  BaseAlignAxisA=+Y  FollAlignAxisB=+Y  BaseAlignAxisB=+Z  RotationStandardAxis=+X  RotationAngle=90  RotationAngleUnits=deg  RotationArbitraryAxis=[0 0 1]  RotationSequenceAxes=FollowerAxes  RotationSequence=XYX  RotationSequenceAngles=[0 0 0]  RotationSequenceAnglesUnits=deg  RotationMatrix=[1 0 0; 0 1 0; 0 0 1]  Quaternion=[1 0 0 0]  TranslationMethod=Cartesian  TranslationCartesianOffset=[0 0 lower_leg_length/2]  TranslationCartesianOffsetUnits=cm  TranslationStandardAxis=+Z  TranslationStandardOffset=0  TranslationStandardOffsetUnits=cm  TranslationROffset=0  TranslationROffsetUnits=m  TranslationThetaOffset=0  TranslationThetaOffsetUnits=deg  TranslationZOffset=0  TranslationZOffsetUnits=m
  Package Measurements : walkingRobotUtils/Package  Measurements 2D  SystemSampleTime=-1  VariantActivationTime=update diagram  AllowFlexibleInterface=on  Latency=0  AutoFrameSizeCalculation=off
  Upper Leg : sm_lib/Body Elements/Cylindrical Solid  CylinderRadius=leg_radius  CylinderRadiusUnits=cm  CylinderLength=upper_leg_length  CylinderLengthUnits=cm  ExportEntireGeometry=off  InertiaType=CalculateFromGeometry  BasedOnType=Density  Density=density  DensityUnits=kg/m^3  Mass=1  MassUnits=kg  CenterOfMass=[0 0 0]  CenterOfMassUnits=m  MomentsOfInertia=[1 1 1]  MomentsOfInertiaUnits=kg*m^2  ProductsOfInertia=[1 1 1]  ProductsOfInertiaUnits=kg*m^2  GraphicType=FromGeometry  MarkerShape=Sphere  MarkerSize=10  GraphicVisPropType=SimpleVisualProperties  GraphicDiffuseColor=[1.0 0.4 0.4]  GraphicOpacity=1.0  GraphicSpecularColor=[0.5 0.5 0.5 1.0]  GraphicAmbientColor=[0.15 0.15 0.15 1.0]  GraphicEmissiveColor=[0.0 0.0 0.0 1.0]  GraphicShininess=75  DoExposeReferenceFrame=on  SerializedFrames=<Frames/>
  Upper Leg to Hip : sm_lib/Frames and Transforms/Rigid Transform  RotationMethod=StandardAxis  FollAlignAxisA=+X  BaseAlignAxisA=+Y  FollAlignAxisB=+Y  BaseAlignAxisB=+Z  RotationStandardAxis=+X  RotationAngle=90  RotationAngleUnits=deg  RotationArbitraryAxis=[0 0 1]  RotationSequenceAxes=FollowerAxes  RotationSequence=XYX  RotationSequenceAngles=[0 0 0]  RotationSequenceAnglesUnits=deg  RotationMatrix=[1 0 0; 0 1 0; 0 0 1]  Quaternion=[1 0 0 0]  TranslationMethod=Cartesian  TranslationCartesianOffset=[0 0 upper_leg_length/2]  TranslationCartesianOffsetUnits=cm  TranslationStandardAxis=+Z  TranslationStandardOffset=0  TranslationStandardOffsetUnits=cm  TranslationROffset=0  TranslationROffsetUnits=m  TranslationThetaOffset=0  TranslationThetaOffsetUnits=deg  TranslationZOffset=0  TranslationZOffsetUnits=m
  G : PMIOPort  Side=Right
  H : PMIOPort  Port=2  Side=Right
  meas : Outport  VectorParamsAs1DForOutWhenUnconnected=off
  wires:
  Foot and Contact/1 -> Package Measurements/1
  Foot and Contact/2 -> Package Measurements/2
  Demux/3 -> Hip Joint/1
  Demux/2 -> Knee Joint/1
  Demux/1 -> Ankle Joint/1
  Ankle Joint/1 -> Package Measurements/3
  Knee Joint/1 -> Package Measurements/4
  Hip Joint/1 -> Package Measurements/5
  torques/1 -> Demux/1
  Package Measurements/1 -> meas/1
  connections:
  G/RConn1 -- Foot and Contact/LConn1
  Foot and Contact/RConn1 -- Foot Offset/LConn1
  Hip Joint/LConn1 -- Upper Leg to Hip/RConn1
  Ankle Joint/LConn1 -- Foot Offset/RConn1
  Hip Joint/RConn1 -- Hip to World Coords/LConn1
  Ankle Joint/RConn1 -- Ankle to Lower Leg/LConn1
  Knee to Upper Leg/LConn1 -- Knee Joint/RConn1
  Ankle to Lower Leg/RConn1 -- Lower Leg/RConn1 -- Lower Leg to Knee/LConn1
  Upper Leg to Hip/LConn1 -- Upper Leg/RConn1 -- Knee to Upper Leg/RConn1
  Knee Joint/LConn1 -- Lower Leg to Knee/RConn1
  H/RConn1 -- Hip to World Coords/RConn1

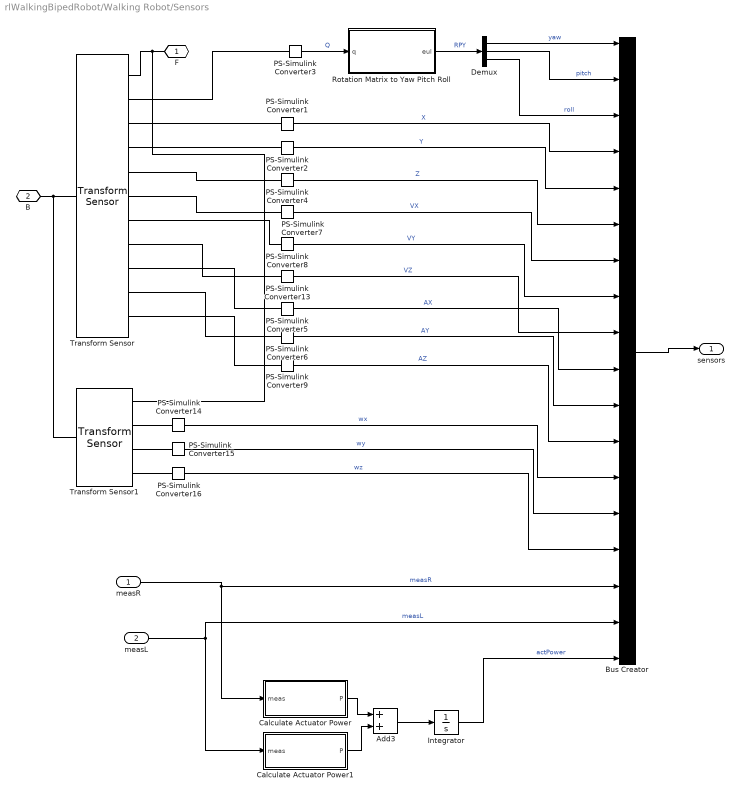
== system rlWalkingBipedRobot/Walking Robot/Sensors ==
  measR : Inport
  measL : Inport  Port=2
  Add3 : Sum
  Bus Creator : BusCreator  Inputs=18
  Calculate Actuator Power : Subsystem
  Calculate Actuator Power1 : Subsystem
  Demux : Demux  Outputs=3
  Integrator : Integrator
  PS-Simulink Converter{1..9,13..16} (13 alike) : nesl_utility/PS-Simulink Converter  PhysicalDomain=network_engine_domain  SubClassName=ps_output  LeftPortType=input  RightPortType=output  PseudoPeriodic=off  Frequencies=[]  VectorFormat=1-D array  Unit=1  AffineConversion=off
  Rotation Matrix to Yaw Pitch Roll : MATLAB Function  TreatAsAtomicUnit=on
  Transform Sensor : sm_lib/Frames and Transforms/Transform Sensor  MeasurementFrame=World  RotationSequence=XYX  SenseAngle=off  SenseAxis=off  SenseQ=on  SenseR=off  SenseRotationSequence=off  SenseOmegaX=off  SenseOmegaY=off  SenseOmegaZ=off  SenseOmega=off  SenseQDot=off  SenseRDot=off  SenseRotationSequenceDot=off  SenseAlphaX=off  SenseAlphaY=off  SenseAlphaZ=off  SenseAlpha=off  SenseQDDot=off  SenseRDDot=off  SenseX=on  SenseY=on  SenseZ=on  SenseXYZ=off  SenseRad=off  SenseAzim=off  SenseDist=off  SenseInc=off  SenseXDot=on  SenseYDot=on  SenseZDot=on  SenseXYZDot=off  SenseRadDot=off  SenseAzimDot=off  SenseDistDot=off  SenseIncDot=off  SenseXDDot=on  SenseYDDot=on  SenseZDDot=on  SenseXYZDDot=off  SenseRadDDot=off  SenseAzimDDot=off  SenseDistDDot=off  SenseIncDDot=off
  Transform Sensor1 : sm_lib/Frames and Transforms/Transform Sensor  MeasurementFrame=NonRotatingFollower  RotationSequence=XYX  SenseAngle=off  SenseAxis=off  SenseQ=off  SenseR=off  SenseRotationSequence=off  SenseOmegaX=on  SenseOmegaY=on  SenseOmegaZ=on  SenseOmega=off  SenseQDot=off  SenseRDot=off  SenseRotationSequenceDot=off  SenseAlphaX=off  SenseAlphaY=off  SenseAlphaZ=off  SenseAlpha=off  SenseQDDot=off  SenseRDDot=off  SenseX=off  SenseY=off  SenseZ=off  SenseXYZ=off  SenseRad=off  SenseAzim=off  SenseDist=off  SenseInc=off  SenseXDot=off  SenseYDot=off  SenseZDot=off  SenseXYZDot=off  SenseRadDot=off  SenseAzimDot=off  SenseDistDot=off  SenseIncDot=off  SenseXDDot=off  SenseYDDot=off  SenseZDDot=off  SenseXYZDDot=off  SenseRadDDot=off  SenseAzimDDot=off  SenseDistDDot=off  SenseIncDDot=off
  F : PMIOPort  Side=Right
  B : PMIOPort  Port=2  Side=Left
  sensors : Outport  VectorParamsAs1DForOutWhenUnconnected=off
  wires:
  PS-Simulink Converter2/1 -> Bus Creator/5  "Y"
  PS-Simulink Converter4/1 -> Bus Creator/6  "Z"
  PS-Simulink Converter5/1 -> Bus Creator/10  "AX"
  Bus Creator/1 -> sensors/1
  PS-Simulink Converter3/1 -> Rotation Matrix to Yaw Pitch Roll/1(q)  "Q"
  PS-Simulink Converter1/1 -> Bus Creator/4  "X"
  PS-Simulink Converter6/1 -> Bus Creator/11  "AY"
  PS-Simulink Converter7/1 -> Bus Creator/7  "VX"
  PS-Simulink Converter8/1 -> Bus Creator/8  "VY"
  PS-Simulink Converter9/1 -> Bus Creator/12  "AZ"
  PS-Simulink Converter13/1 -> Bus Creator/9  "VZ"
  Rotation Matrix to Yaw Pitch Roll/1(eul) -> Demux/1  "RPY"
  Demux/3 -> Bus Creator/3  "roll"
  Demux/2 -> Bus Creator/2  "pitch"
  Demux/1 -> Bus Creator/1  "yaw"
  PS-Simulink Converter14/1 -> Bus Creator/13  "wx"
  PS-Simulink Converter15/1 -> Bus Creator/14  "wy"
  PS-Simulink Converter16/1 -> Bus Creator/15  "wz"
  measR/1 -> Calculate Actuator Power/1(meas), Bus Creator/16  "measR"
  measL/1 -> Calculate Actuator Power1/1(meas), Bus Creator/17  "measL"
  Calculate Actuator Power/1(P) -> Add3/1
  Calculate Actuator Power1/1(P) -> Add3/2
  Add3/1 -> Integrator/1
  Integrator/1 -> Bus Creator/18  "actPower"
  connections:
  PS-Simulink Converter1/LConn1 -- Transform Sensor/RConn3
  PS-Simulink Converter3/LConn1 -- Transform Sensor/RConn2
  Transform Sensor/RConn1 -- Transform Sensor1/RConn1 -- F/RConn1
  Transform Sensor/RConn5 -- PS-Simulink Converter4/LConn1
  Transform Sensor/RConn4 -- PS-Simulink Converter2/LConn1
  Transform Sensor/LConn1 -- Transform Sensor1/LConn1 -- B/RConn1
  PS-Simulink Converter7/LConn1 -- Transform Sensor/RConn6
  PS-Simulink Converter14/LConn1 -- Transform Sensor1/RConn2
  PS-Simulink Converter15/LConn1 -- Transform Sensor1/RConn3
  Transform Sensor1/RConn4 -- PS-Simulink Converter16/LConn1
  Transform Sensor/RConn7 -- PS-Simulink Converter8/LConn1
  PS-Simulink Converter13/LConn1 -- Transform Sensor/RConn8
  PS-Simulink Converter5/LConn1 -- Transform Sensor/RConn9
  Transform Sensor/RConn10 -- PS-Simulink Converter6/LConn1
  PS-Simulink Converter9/LConn1 -- Transform Sensor/RConn11

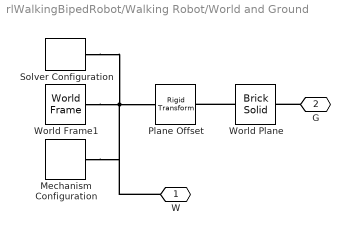
== system rlWalkingBipedRobot/Walking Robot/World and Ground ==
  Mechanism Configuration : sm_lib/Utilities/Mechanism Configuration  UniformGravity=Constant  GravityVector=[0 0 -9.80665]  GravityVectorUnits=m/s^2  LinearizationDelta=0.001  JointModeTransitionNonlinearIterations=2
  Plane Offset : sm_lib/Frames and Transforms/Rigid Transform  RotationMethod=None  FollAlignAxisA=+X  BaseAlignAxisA=+Y  FollAlignAxisB=+Y  BaseAlignAxisB=+Z  RotationStandardAxis=+Z  RotationAngle=0.0  RotationAngleUnits=deg  RotationArbitraryAxis=[0 0 1]  RotationSequenceAxes=FollowerAxes  RotationSequence=XYX  RotationSequenceAngles=[0 0 0]  RotationSequenceAnglesUnits=deg  RotationMatrix=[1 0 0; 0 1 0; 0 0 1]  Quaternion=[1 0 0 0]  TranslationMethod=StandardAxis  TranslationCartesianOffset=[0 0 0]  TranslationCartesianOffsetUnits=m  TranslationStandardAxis=-Z  TranslationStandardOffset=height_plane/2  TranslationStandardOffsetUnits=m  TranslationROffset=0  TranslationROffsetUnits=m  TranslationThetaOffset=0  TranslationThetaOffsetUnits=deg  TranslationZOffset=0  TranslationZOffsetUnits=m
  Solver Configuration : nesl_utility/Solver Configuration  PhysicalDomain=network_engine_domain  SubClassName=solver  LeftPortType=input  RightPortType=generic  Tones=[]  Harmonics=[]  SimulateNoise=off  Profile=off  UseLocalSampling=off  EnableSwitchedLinearOptims=on  FrequencyDomain=off  UseCCode=off  RelTol=0.001  AbsTol=1e-06  MinStep=1e-09  ToWorkspace=off  RevertToSquareIcSolve=off  NumHomotopyIterations=100  PhasorMode=off  PhasorModeNumHarmonics=1  ConsistencySolver=NEWTON_FTOL  IndexReductionMethod=DerivativeReplacement  DoDC=off  ResidualTolerance=1e-09  ConsistencyTolSource=GLOBAL  ConsistencyAbsTol=0.001  ConsistencyRelTol=0.001  ConsistencyTolFactor=0.001  UseLocalSolver=off  LocalSolverChoice=NE_TRAPEZOIDAL_ADVANCER  ResolveIndetEquations=on  FunctionEvalNumThread=1  LocalSolverSampleTime=Ts  DoFixedCost=off  MaxNonlinIter=3  MaxModeIter=2  ComputeImpulses=off  ImpulseIterations=2  LinearAlgebra=Sparse  LinearAlgebraNumThread=0  EquationFormulation=NE_TIME_EF  DelaysMemoryBudget=1024  AutomaticFiltering=on  FilteringTimeConstant=0.001  PartitionStorageMethod=AS_NEEDED  PartitionMemoryBudget=1024  PartitionMethod=FAST  MultibodyUseLocalSolver=off  MultibodyLocalSolverChoice=ODE1  MultibodyLocalSolverSampleTime=0.001
  World Frame1 : sm_lib/Frames and Transforms/World Frame
  World Plane : sm_lib/Body Elements/Brick Solid  BrickDimensions="[plane_x plane_y  height_plane]"  BrickDimensionsUnits=m  ExportEntireGeometry=on  InertiaType=CalculateFromGeometry  BasedOnType=Density  Density=density  DensityUnits=kg/(m^3)  Mass=1  MassUnits=kg  CenterOfMass=[0 0 0]  CenterOfMassUnits=m  MomentsOfInertia=[1 1 1]  MomentsOfInertiaUnits=kg*m^2  ProductsOfInertia=[0 0 0]  ProductsOfInertiaUnits=kg*m^2  GraphicType=FromGeometry  MarkerShape=Sphere  MarkerSize=10  GraphicVisPropType=SimpleVisualProperties  GraphicDiffuseColor=[1.0 1.0 0.8]  GraphicOpacity=0.5  GraphicSpecularColor=[0.5 0.5 0.5 1.0]  GraphicAmbientColor=[0.15 0.15 0.15 1.0]  GraphicEmissiveColor=[0.0 0.0 0.0 1.0]  GraphicShininess=75  DoExposeReferenceFrame=on  SerializedFrames=<Frames/>
  W : PMIOPort  Side=Left
  G : PMIOPort  Port=2  Side=Right
  connections:
  G/RConn1 -- World Plane/LConn1
  World Plane/RConn1 -- Plane Offset/RConn1
  Solver Configuration/RConn1 -- Plane Offset/LConn1 -- Mechanism Configuration/RConn1 -- W/RConn1 -- World Frame1/RConn1

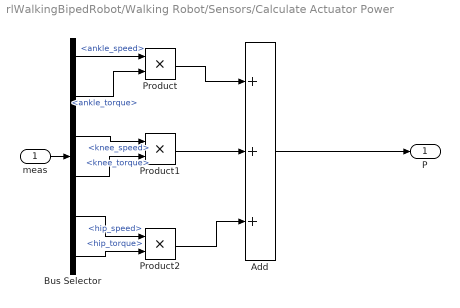
== system rlWalkingBipedRobot/Walking Robot/Sensors/Calculate Actuator Power ==
  meas : Inport
  Add : Sum  Inputs=3
  Bus Selector : BusSelector  OutputSignals=ankle_speed,ankle_torque,knee_speed,knee_torque,hip_speed,hip_torque
  Product : Product
  Product1 : Product
  Product2 : Product
  P : Outport  VectorParamsAs1DForOutWhenUnconnected=off
  wires:
  meas/1 -> Bus Selector/1
  Product2/1 -> Add/3
  Product1/1 -> Add/2
  Product/1 -> Add/1
  Add/1 -> P/1
  Bus Selector/1 -> Product/1  "<ankle_speed>"
  Bus Selector/2 -> Product/2  "<ankle_torque>"
  Bus Selector/3 -> Product1/1  "<knee_speed>"
  Bus Selector/4 -> Product1/2  "<knee_torque>"
  Bus Selector/5 -> Product2/1  "<hip_speed>"
  Bus Selector/6 -> Product2/2  "<hip_torque>"

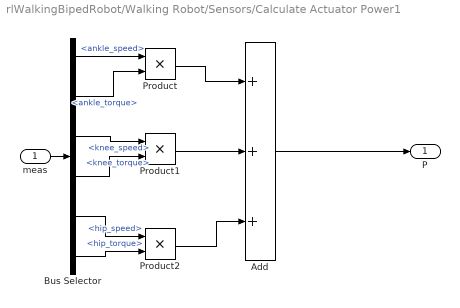
== system rlWalkingBipedRobot/Walking Robot/Sensors/Calculate Actuator Power1 ==
  meas : Inport
  Add : Sum  Inputs=3
  Bus Selector : BusSelector  OutputSignals=ankle_speed,ankle_torque,knee_speed,knee_torque,hip_speed,hip_torque
  Product : Product
  Product1 : Product
  Product2 : Product
  P : Outport  VectorParamsAs1DForOutWhenUnconnected=off
  wires:
  Bus Selector/6 -> Product2/2  "<hip_torque>"
  Bus Selector/5 -> Product2/1  "<hip_speed>"
  Bus Selector/4 -> Product1/2  "<knee_torque>"
  Bus Selector/3 -> Product1/1  "<knee_speed>"
  Bus Selector/2 -> Product/2  "<ankle_torque>"
  Bus Selector/1 -> Product/1  "<ankle_speed>"
  Add/1 -> P/1
  Product/1 -> Add/1
  Product1/1 -> Add/2
  Product2/1 -> Add/3
  meas/1 -> Bus Selector/1

== matlab function rlWalkingBipedRobot/Walking Robot/Sensors/Rotation Matrix to Yaw Pitch Roll ==
  data: q input; eul output
function eul = calcAttitude(q)

% Normalize the quaternions
q = bsxfun(@times, q, 1./sqrt(sum(q.^2,1)));
qw = q(1);
qx = q(2);
qy = q(3);
qz = q(4);

% Pre-allocate output
eul = zeros(3, 1, 'like', q);

aSinInput = -2*(qx.*qz-qw.*qy);
aSinInput(aSinInput > 1) = 1;
aSinInput(aSinInput < -1) = -1;

eul = [ atan2( 2*(qx.*qy+qw.*qz), qw.^2 + qx.^2 - qy.^2 - qz.^2 ); ...
    asin( aSinInput ); ...
    atan2( 2*(qy.*qz+qw.*qx), qw.^2 - qx.^2 - qy.^2 + qz.^2 )];
